simulink model "EINT_RL_closed_loop_x"  (R2025a)
settings: Solver=FixedStepAuto  StartTime=0.0  StopTime=T_end  FixedStep=Ts  RelTol=1e-3
values from neighbouring files (symbols this model uses):
  Ts = 0.05    [EINT_RL_eval_follow.m]    (also in EINT_RL_eval_x.m; rl_controller_follow.m; rl_controller_full_x.m)
settings Model: Creator=PC-Ali  LastModifiedBy=PC-Ali

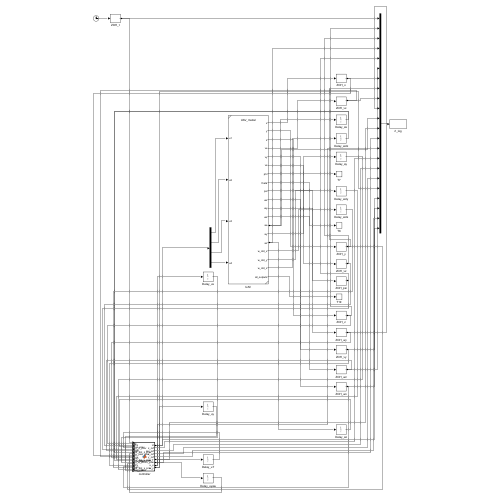
[thumbnail: Simulink's stored preview of the top-level diagram]
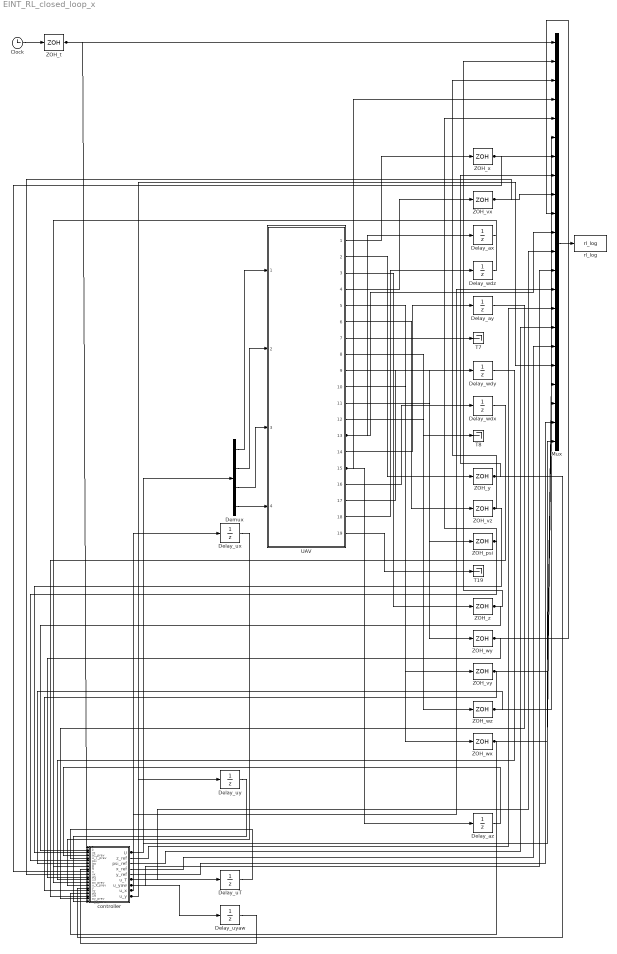
== system EINT_RL_closed_loop_x ==
  Clock : Clock
  Delay_ax : UnitDelay  SampleTime=Ts  HasFrameUpgradeWarning=on
  Delay_ay : UnitDelay  SampleTime=Ts  HasFrameUpgradeWarning=on
  Delay_az : UnitDelay  SampleTime=Ts  HasFrameUpgradeWarning=on
  Delay_uT : UnitDelay  SampleTime=Ts  HasFrameUpgradeWarning=on
  Delay_ux : UnitDelay  SampleTime=Ts  HasFrameUpgradeWarning=on
  Delay_uy : UnitDelay  SampleTime=Ts  HasFrameUpgradeWarning=on
  Delay_uyaw : UnitDelay  SampleTime=Ts  HasFrameUpgradeWarning=on
  Delay_wdx : UnitDelay  SampleTime=Ts  HasFrameUpgradeWarning=on
  Delay_wdy : UnitDelay  SampleTime=Ts  HasFrameUpgradeWarning=on
  Delay_wdz : UnitDelay  SampleTime=Ts  HasFrameUpgradeWarning=on
  Demux : Demux
  Mux : Mux  Inputs=22
  T19 : Terminator
  T7 : Terminator
  T8 : Terminator
  UAV : Subsystem  ReferencedSubsystem=UAV_model
  ZOH_psi : ZeroOrderHold  SampleTime=Ts
  ZOH_t : ZeroOrderHold  SampleTime=Ts
  ZOH_vx : ZeroOrderHold  SampleTime=Ts
  ZOH_vy : ZeroOrderHold  SampleTime=Ts
  ZOH_vz : ZeroOrderHold  SampleTime=Ts
  ZOH_wx : ZeroOrderHold  SampleTime=Ts
  ZOH_wy : ZeroOrderHold  SampleTime=Ts
  ZOH_wz : ZeroOrderHold  SampleTime=Ts
  ZOH_x : ZeroOrderHold  SampleTime=Ts
  ZOH_y : ZeroOrderHold  SampleTime=Ts
  ZOH_z : ZeroOrderHold  SampleTime=Ts
  controller : MATLAB Function  TreatAsAtomicUnit=on
  rl_log : ToWorkspace  VariableName=rl_log  SampleTime=Ts
  wires:
  controller/5(y_ref) -> Mux/21
  controller/3(psi_ref) -> Mux/16
  controller/9(u_y) -> Mux/18, Delay_uy/1
  Clock/1 -> ZOH_t/1
  controller/6(u_T) -> Mux/12, Delay_uT/1
  controller/4(x_ref) -> Mux/17
  controller/2(z_ref) -> Mux/15
  controller/8(u_x) -> Mux/14, Delay_ux/1
  ZOH_t/1 -> Mux/1, controller/1(t)
  controller/1(U) -> Mux/22, Demux/1
  controller/7(u_yaw) -> Mux/13, Delay_uyaw/1
  Demux/1 -> UAV/1
  Demux/2 -> UAV/2
  Demux/3 -> UAV/3
  Demux/4 -> UAV/4
  ZOH_wz/1 -> Mux/6, controller/7(wz)
  UAV/13 -> Mux/11, Delay_ax/1
  Delay_ux/1 -> controller/15(u_x_prev)
  ZOH_x/1 -> controller/10(x), Mux/7
  UAV/14 -> Delay_ay/1
  Delay_uy/1 -> controller/21(u_y_prev)
  ZOH_vz/1 -> controller/3(vz), Mux/3
  UAV/15 -> Mux/4, Delay_az/1
  Delay_uT/1 -> controller/5(u_T_prev)
  ZOH_psi/1 -> controller/6(psi), Mux/5
  UAV/16 -> Delay_wdx/1
  Delay_uyaw/1 -> controller/9(u_yaw_prev)
  Delay_wdx/1 -> controller/19(w_dot_x_prev)
  UAV/17 -> Delay_wdy/1
  UAV/1 -> ZOH_x/1
  ZOH_z/1 -> controller/2(z), Mux/2
  Delay_ay/1 -> controller/20(ay_prev)
  UAV/18 -> Delay_wdz/1
  UAV/2 -> ZOH_y/1
  Delay_wdy/1 -> controller/13(w_dot_y_prev)
  UAV/19 -> T19/1
  UAV/3 -> ZOH_z/1
  Delay_ax/1 -> controller/14(ax_prev)
  UAV/4 -> ZOH_vx/1
  Delay_az/1 -> controller/4(az_prev)
  UAV/5 -> ZOH_vy/1
  Delay_wdz/1 -> controller/8(w_dot_z_prev)
  UAV/6 -> ZOH_vz/1
  ZOH_wx/1 -> Mux/20, controller/18(wx)
  UAV/7 -> T7/1
  UAV/8 -> T8/1
  ZOH_y/1 -> controller/16(y), Mux/8
  UAV/9 -> ZOH_psi/1
  ZOH_vy/1 -> controller/17(vy), Mux/19
  UAV/10 -> ZOH_wx/1
  ZOH_vx/1 -> controller/11(vx), Mux/9
  UAV/11 -> ZOH_wy/1
  ZOH_wy/1 -> Mux/10, controller/12(wy)
  UAV/12 -> ZOH_wz/1
  Mux/1 -> rl_log/1

== matlab function EINT_RL_closed_loop_x/controller ==
  data: t input; U output; z input; vz input; az_prev input; u_T_prev input; psi input; wz input; w_dot_z_prev input; u_yaw_prev input; x input; vx input; wy input; w_dot_y_prev input; ax_prev input; u_x_prev input; y input; vy input; wx input; w_dot_x_prev input; ay_prev input; u_y_prev input; z_ref output; psi_ref output; x_ref output; y_ref output; u_T output; u_yaw output; u_x output; u_y output
function [U, z_ref, psi_ref, x_ref, y_ref, u_T, u_yaw, u_x, u_y] = controller(t, z, vz, az_prev, u_T_prev, psi, wz, w_dot_z_prev, u_yaw_prev, x, vx, wy, w_dot_y_prev, ax_prev, u_x_prev, y, vy, wx, w_dot_x_prev, ay_prev, u_y_prev)
coder.extrinsic('rl_controller_full_x');
U = zeros(4, 1); z_ref = 0; psi_ref = 0; x_ref = 0; y_ref = 0; u_T = 0; u_yaw = 0; u_x = 0; u_y = 0;
[U, z_ref, psi_ref, x_ref, y_ref, u_T, u_yaw, u_x, u_y] = rl_controller_full_x(t, z, vz, az_prev, u_T_prev, psi, wz, w_dot_z_prev, u_yaw_prev, x, vx, wy, w_dot_y_prev, ax_prev, u_x_prev, y, vy, wx, w_dot_x_prev, ay_prev, u_y_prev);
